simulink model "WallModel"  (R2024a)
settings: Solver=daessc  StartTime=0.0  StopTime=12*3600  FixedStep=3600  MaxStep=3  RelTol=1e-3  AbsTol=1e-3
PreLoadFcn:
  | WallModelParams
values from neighbouring files (symbols this model uses):
  roomHeight = 5    [WallModelParams.m]
undefined symbols (not defined in the file or in its folder): flow, wall, win
libraries: fl_lib x67, nesl_utility x2
CloseFcn:
  | clear flow out roomHeight wall win
settings Model: Creator=vikrants  LastModifiedBy=vikrants
settings SolverCC: AutoScaleAbsTol=off  AlgebraicLoopSolver=TrustRegion  MaxZcPerStep=1
settings DebuggingCC: UnconnectedInputMsg=warning  UnconnectedOutputMsg=warning  UnconnectedLineMsg=warning  SymbolicDimsDataTypeCodeGenerationDiagnostic=none
settings ModelReferenceCC: EnableRefExpFcnMdlSchedulingChecks=on
settings SFSimCC: CustomCodeUndefinedFunction=UseInterfaceOnly
settings RTWCC: GPUComputeCapability=3.5  DLArmComputeVersion=19.05
settings SimscapeCC: SimscapeLogType=all  SimscapeLogSimulationStatistics=on  SimscapeLogDataHistory=10000

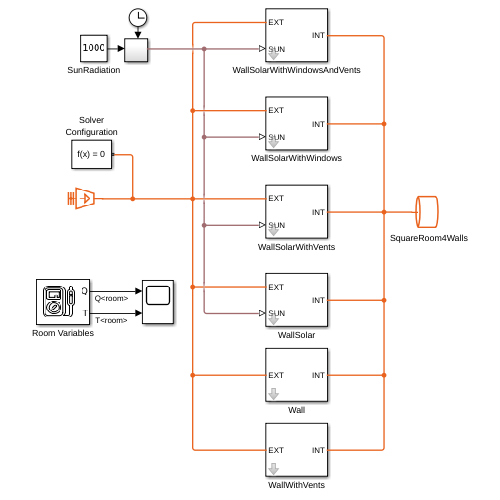
[thumbnail: Simulink's stored preview of the top-level diagram]
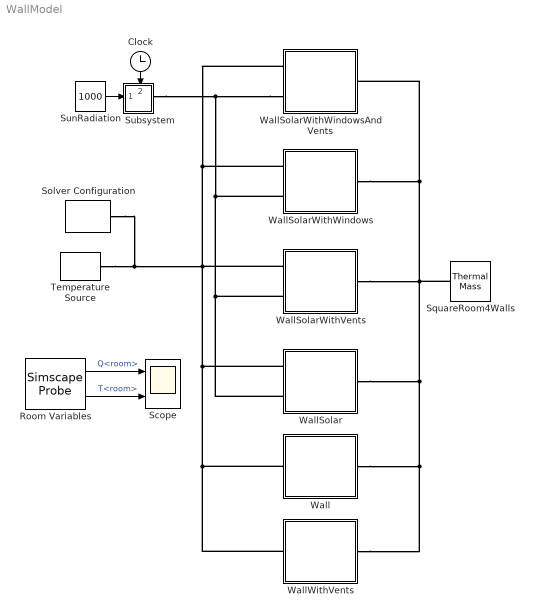
== system WallModel ==
  Clock : Clock
  Room Variables : SimscapeProbe  BoundBlock=26  Variables={Q, T}
  Scope : Scope  NumInputPorts=2
  Solver Configuration : nesl_utility/Solver Configuration  PhysicalDomain=network_engine_domain  SubClassName=solver  LeftPortType=input  RightPortType=generic  Tones=[]  Harmonics=[]  SimulateNoise=off  Profile=off  UseLocalSampling=off  EnableSwitchedLinearOptims=on  FrequencyDomain=off  UseCCode=off  RelTol=0.001  AbsTol=1e-06  MinStep=1e-09  ToWorkspace=off  RevertToSquareIcSolve=off  NumHomotopyIterations=100  PhasorMode=off  PhasorModeNumHarmonics=1  ConsistencySolver=NEWTON_XTOL_AFTER_FTOL  IndexReductionMethod=DerivativeReplacement  DoDC=off  ResidualTolerance=1e-09  ConsistencyTolSource=GLOBAL  ConsistencyAbsTol=0.001  ConsistencyRelTol=0.001  ConsistencyTolFactor=0.001  UseLocalSolver=off  LocalSolverChoice=NE_BACKWARD_EULER_ADVANCER  ResolveIndetEquations=on  FunctionEvalNumThread=1  LocalSolverSampleTime=0.001  DoFixedCost=off  MaxNonlinIter=3  MaxModeIter=2  ComputeImpulses=off  ImpulseIterations=2  LinearAlgebra=auto  LinearAlgebraNumThread=0  EquationFormulation=NE_TIME_EF  DelaysMemoryBudget=1024  AutomaticFiltering=on  FilteringTimeConstant=0.001  PartitionStorageMethod=AS_NEEDED  PartitionMemoryBudget=1024  PartitionMethod=ROBUST  MultibodyUseLocalSolver=off  MultibodyLocalSolverChoice=ODE1  MultibodyLocalSolverSampleTime=0.001
  SquareRoom4Walls : fl_lib/Thermal/Thermal Elements/Thermal Mass  mass_type=foundation.enum.constant_variable.constant  mass=((wall.area+win.area)/roomHeight)^2*flow.airDen kg  sp_heat=flow.airCp J/(K*kg)  mass_min=1e-6 kg  num_ports=foundation.enum.numPorts2.one  m_specify=off  m_priority=High  m=1 kg  m_nominal_specify=off  m_nominal_value=1  m_nominal_unit=kg  T_specify=on  T_priority=High  T=flow.iniT K  T_nominal_specify=off  T_nominal_value=1  T_nominal_unit=K  Q_specify=off  Q_priority=None  Q=0 W  Q_nominal_specify=off  Q_nominal_value=1  Q_nominal_unit=W
  Subsystem : Subsystem
      settings: PortSchema="{\"entries\":[{\"content\":{\"sides\":[{\"content\":{\"connectorIds\":[\"In1\"]},\"type\":\"ConnectorPlacement.EquallySpacedRectSide\",\"uuid\":\"3d46a215-694f-4d20-bc42-8059ad6c23bd\"},{\"content\":{\"connectorIds\":[\"RConn1\"],\"side\":\"RIGHT\"},\"type\":\"ConnectorPlacement.EquallySpacedRectSide\",\"uuid\":\"4734f55e-0044-4fb6-ae62-80969ebadacf\"},{\"content\":{\"connectorIds\":[\"In2\"],\"side\":\"TOP\"},\"type\":\"ConnectorPlacement.EquallySpacedRectSide\",\"uuid\":\"f13755de-7156-4054-ad92-dbe96d889caf\"}]},\"type\":\"ConnectorPlacement.EquallySpacedConnector\",\"uuid\":\"e23b6fdc-de89-4593-96e6-8ffafb2d38ae\"}],\"packageUris\":[\"http://schema.mathworks.com/mf0/Connector/R2020b\"],\"version\":\"1.0\"}"
  SunRadiation : Constant  Value=1000
  Temperature Source : fl_lib/Thermal/Thermal Sources/Temperature Source  temperature=300 K
  Wall : Subsystem  mask{wallArea=wall.area, wallThickness=wall.thickness, wallMaterialMass=wall.mass, wallMaterialCp=wall.Cp, wallThermalK=wall.K, wallAbsorptivity=wall.absorp, extToWallHTC=flow.htc.ext, intToRoomHTC=flow.htc.int, wallTemperature=flow.iniT}
      mask prompts: wallArea "Wall area"; wallThickness "Wall thickness"; wallMaterialMass "Wall material mass"; wallMaterialCp "Wall material heat capacity"; wallThermalK "Wall thermal conductivity"; wallAbsorptivity "Wall absorptivity"; extToWallHTC "Effective heat transfer coefficient from ambient to wall surface"; intToRoomHTC "Effective heat transfer coefficient from internal surface to the room"; wallTemperature "Wall initial temperature"
      mask DialogControl DescTextVar Prompt: Use this custom component to specify the wall heat transfer into a room.
      mask DialogControl Parameters Prompt: Parameters
  WallSolar : Subsystem  mask{wallArea=wall.area, wallThickness=wall.thickness, wallMaterialMass=wall.mass, wallMaterialCp=wall.Cp, wallThermalK=wall.K, wallAbsorptivity=wall.absorp, extToWallHTC=flow.htc.ext, intToRoomHTC=flow.htc.int, wallTemperature=flow.iniT}
      mask prompts: wallArea "Wall area"; wallThickness "Wall thickness"; wallMaterialMass "Wall material mass"; wallMaterialCp "Wall material heat capacity"; wallThermalK "Wall thermal conductivity"; wallAbsorptivity "Wall absorptivity"; extToWallHTC "Effective heat transfer coefficient from ambient to wall surface"; intToRoomHTC "Effective heat transfer coefficient from internal surface to the room"; wallTemperature "Wall initial temperature"
      mask DialogControl DescTextVar Prompt: Use this custom component to specify the wall heat transfer into a room.
      mask DialogControl Parameters Prompt: Parameters
  WallSolarWithVents : Subsystem  mask{wallArea=wall.area, wallThickness=wall.thickness, wallMaterialMass=wall.mass, wallMaterialCp=wall.Cp, wallThermalK=wall.K, wallAbsorptivity=wall.absorp, ventArea=flow.vent.area, extToWallHTC=flow.htc.ext, intToRoomHTC=flow.htc.int, wallTemperature=flow.iniT}
      mask prompts: wallArea "Wall area"; wallThickness "Wall thickness"; wallMaterialMass "Wall material mass"; wallMaterialCp "Wall material heat capacity"; wallThermalK "Wall thermal conductivity"; wallAbsorptivity "Wall absorptivity"; ventArea "Vent area"; extToWallHTC "Effective heat transfer coefficient from ambient to wall surface"; intToRoomHTC "Effective heat transfer coefficient from internal surface to the room"; wallTemperature "Wall initial temperature"
      mask DialogControl DescTextVar Prompt: Use this custom component to specify the wall and assicated heat transfer into a room. You must specify the wall and window material properties along with the vent size.
      mask DialogControl Parameters Prompt: Parameters
  WallSolarWithWindows : Subsystem  mask{winArea=win.area, winThickness=win.thickness, winMaterialMass=win.mass, winMaterialCp=win.Cp, winThermalK=win.K, winAbsorptivity=win.absorp, winTransmissivity=win.trans, wallArea=wall.area, wallThickness=wall.thickness, wallMaterialMass=wall.mass, wallMaterialCp=wall.Cp, wallThermalK=wall.K, wallAbsorptivity=wall.absorp, extToWallHTC=flow.htc.ext, intToRoomHTC=flow.htc.int, wallTemperature=flow.iniT, winTemperature=flow.iniT}
      mask prompts: winArea "Window area"; winThickness "Window thickness"; winMaterialMass "Window material mass"; winMaterialCp "Window material heat capacity"; winThermalK "Window thermal conductivity"; winAbsorptivity "Window Absorptivity"; winTransmissivity "Window transmissivity"; wallArea "Wall area"; wallThickness "Wall thickness"; wallMaterialMass "Wall material mass"; wallMaterialCp "Wall material heat capacity"; wallThermalK "Wall thermal conductivity"; wallAbsorptivity "Wall absorptivity"; extToWallHTC "Effective heat transfer coefficient from ambient to wall surface"; intToRoomHTC "Effective heat transfer coefficient from internal surface to the room"; wallTemperature "Wall initial temperature"; winTemperature "Window initial temperature"
      mask DialogControl DescTextVar Prompt: Use this custom component to specify the wall and assicated heat transfer into a room. You must specify the wall and window material properties.
      mask DialogControl Parameters Prompt: Parameters
  WallSolarWithWindowsAndVents : Subsystem  mask{winArea=win.area, winThickness=win.thickness, winMaterialMass=win.mass, winMaterialCp=win.Cp, winThermalK=win.K, winAbsorptivity=win.absorp, winTransmissivity=win.trans, wallArea=wall.area, wallThickness=wall.thickness, wallMaterialMass=wall.mass, wallMaterialCp=wall.Cp, wallThermalK=wall.K, wallAbsorptivity=wall.absorp, ventArea=flow.vent.area, extToWallHTC=flow.htc.ext, intToRoomHTC=flow.htc.int, wallTemperature=flow.iniT, winTemperature=flow.iniT}
      mask prompts: winArea "Window area"; winThickness "Window thickness"; winMaterialMass "Window material mass"; winMaterialCp "Window material heat capacity"; winThermalK "Window thermal conductivity"; winAbsorptivity "Window Absorptivity"; winTransmissivity "Window transmissivity"; wallArea "Wall area"; wallThickness "Wall thickness"; wallMaterialMass "Wall material mass"; wallMaterialCp "Wall material heat capacity"; wallThermalK "Wall thermal conductivity"; wallAbsorptivity "Wall absorptivity"; ventArea "Vent area"; extToWallHTC "Effective heat transfer coefficient from ambient to wall surface"; intToRoomHTC "Effective heat transfer coefficient from internal surface to the room"; wallTemperature "Wall initial temperature"; winTemperature "Window initial temperature"
      mask DialogControl DescTextVar Prompt: Use this custom component to specify the wall and assicated heat transfer into a room. You must specify the wall and window material properties along with the vent size.
      mask DialogControl Parameters Prompt: Parameters
  WallWithVents : Subsystem  mask{wallArea=wall.area, wallThickness=wall.thickness, wallMaterialMass=wall.mass, wallMaterialCp=wall.Cp, wallThermalK=wall.K, ventArea=flow.vent.area, extToWallHTC=flow.htc.ext, intToRoomHTC=flow.htc.int, wallTemperature=flow.iniT}
      mask prompts: wallArea "Wall area"; wallThickness "Wall thickness"; wallMaterialMass "Wall material mass"; wallMaterialCp "Wall material heat capacity"; wallThermalK "Wall thermal conductivity"; ventArea "Vent area"; extToWallHTC "Effective heat transfer coefficient from ambient to wall surface"; intToRoomHTC "Effective heat transfer coefficient from internal surface to the room"; wallTemperature "Wall initial temperature"
      mask DialogControl DescTextVar Prompt: Use this custom component to specify the wall and assicated heat transfer into a room. You must specify the wall and window material properties along with the vent size.
      mask DialogControl Parameters Prompt: Parameters
  wires:
  Room Variables/2 -> Scope/2  "T<room>"
  Room Variables/1 -> Scope/1  "Q<room>"
  Clock/1 -> Subsystem/2(" ")
  SunRadiation/1 -> Subsystem/1("  ")
  connections:
  SquareRoom4Walls/LConn1 -- WallSolarWithWindowsAndVents/RConn1 -- WallSolarWithWindows/RConn1 -- WallWithVents/RConn1 -- Wall/RConn1 -- WallSolar/RConn1 -- WallSolarWithVents/RConn1
  WallSolarWithWindowsAndVents/LConn2 -- WallSolar/LConn2 -- WallSolarWithVents/LConn2 -- WallSolarWithWindows/LConn2 -- Subsystem/RConn1
  Temperature Source/LConn1 -- Solver Configuration/RConn1 -- WallSolarWithWindowsAndVents/LConn1 -- WallSolarWithWindows/LConn1 -- WallWithVents/LConn1 -- Wall/LConn1 -- WallSolar/LConn1 -- WallSolarWithVents/LConn1

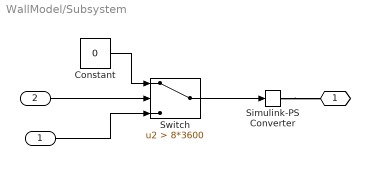
== system WallModel/Subsystem ==
  "  " : Inport
  " " : Inport  Port=2
  Constant : Constant  Value=0
  Simulink-PS Converter : nesl_utility/Simulink-PS Converter  PhysicalDomain=network_engine_domain  SubClassName=ps_input  LeftPortType=input  RightPortType=output  PseudoPeriodic=off  Frequencies=[]  NoiseDistribution=none  NoiseParameters=[]  Unit=W/m^2  AffineConversion=off  FilteringAndDerivatives=filter  SimscapeFilterOrder=1  InputFilterTimeConstant=0.001  UdotUserProvided=0
  Switch : Switch  Criteria=u2 > Threshold  Threshold=8*3600  SaturateOnIntegerOverflow=off  InputSameDT=off
  "   " : PMIOPort  Side=Right
  wires:
  Switch/1 -> Simulink-PS Converter/1
  Constant/1 -> Switch/1
  " "/1 -> Switch/2
  "  "/1 -> Switch/3
  connections:
  Simulink-PS Converter/RConn1 -- "   "/RConn1

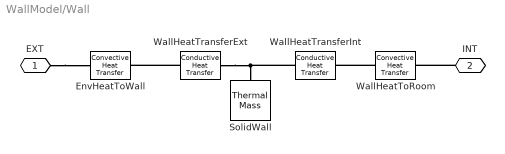
== system WallModel/Wall ==
  EnvHeatToWall : fl_lib/Thermal/Thermal Elements/Convective Heat Transfer  thermal_type=foundation.enum.constant_variable.constant  area=wallArea m^2  heat_tr_coeff=extToWallHTC W/(K*m^2)  min_heat_tr_coeff=1e-3 W/(K*m^2)  T_specify=off  T_priority=None  T=0 K  T_nominal_specify=off  T_nominal_value=1  T_nominal_unit=K  Q_specify=off  Q_priority=None  Q=0 W  Q_nominal_specify=off  Q_nominal_value=1  Q_nominal_unit=W
  SolidWall : fl_lib/Thermal/Thermal Elements/Thermal Mass  mass_type=foundation.enum.constant_variable.constant  mass=wallMaterialMass kg  sp_heat=wallMaterialCp J/(K*kg)  mass_min=1e-6 kg  num_ports=foundation.enum.numPorts2.one  m_specify=off  m_priority=High  m=1 kg  m_nominal_specify=off  m_nominal_value=1  m_nominal_unit=kg  T_specify=on  T_priority=High  T=wallTemperature K  T_nominal_specify=off  T_nominal_value=1  T_nominal_unit=K  Q_specify=off  Q_priority=None  Q=0 W  Q_nominal_specify=off  Q_nominal_value=1  Q_nominal_unit=W
  WallHeatToRoom : fl_lib/Thermal/Thermal Elements/Convective Heat Transfer  thermal_type=foundation.enum.constant_variable.constant  area=wallArea m^2  heat_tr_coeff=intToRoomHTC W/(K*m^2)  min_heat_tr_coeff=1e-3 W/(K*m^2)  T_specify=off  T_priority=None  T=0 K  T_nominal_specify=off  T_nominal_value=1  T_nominal_unit=K  Q_specify=off  Q_priority=None  Q=0 W  Q_nominal_specify=off  Q_nominal_value=1  Q_nominal_unit=W
  WallHeatTransferExt : fl_lib/Thermal/Thermal Elements/Conductive Heat Transfer  thermal_type=foundation.enum.ConstantVariableTabulated.Constant  wall_geometry=foundation.enum.ConductionWallGeometry.Planar  area=wallArea m^2  thickness=wallThickness m  d_in=0.05 m  d_out=0.1 m  L=1 m  th_cond_min=10 W/(K*m)  th_cond=wallThermalK W/(K*m)  th_cond_TLU=[413, 401, 392, 383, 371, 357, 342] W/(K*m)  temp_TLU=[200, 273, 400, 600, 800, 1000, 1200] K  T_specify=off  T_priority=None  T=0 K  T_nominal_specify=off  T_nominal_value=1  T_nominal_unit=K  Q_specify=off  Q_priority=None  Q=0 W  Q_nominal_specify=off  Q_nominal_value=1  Q_nominal_unit=W
  WallHeatTransferInt : fl_lib/Thermal/Thermal Elements/Conductive Heat Transfer  thermal_type=foundation.enum.ConstantVariableTabulated.Constant  wall_geometry=foundation.enum.ConductionWallGeometry.Planar  area=wallArea m^2  thickness=wallThickness m  d_in=0.05 m  d_out=0.1 m  L=1 m  th_cond_min=10 W/(K*m)  th_cond=wallThermalK W/(K*m)  th_cond_TLU=[413, 401, 392, 383, 371, 357, 342] W/(K*m)  temp_TLU=[200, 273, 400, 600, 800, 1000, 1200] K  T_specify=off  T_priority=None  T=0 K  T_nominal_specify=off  T_nominal_value=1  T_nominal_unit=K  Q_specify=off  Q_priority=None  Q=0 W  Q_nominal_specify=off  Q_nominal_value=1  Q_nominal_unit=W
  EXT : PMIOPort  Side=Left
  INT : PMIOPort  Port=2  Side=Right
  connections:
  WallHeatToRoom/LConn1 -- WallHeatTransferInt/RConn1
  INT/RConn1 -- WallHeatToRoom/RConn1
  EXT/RConn1 -- EnvHeatToWall/LConn1
  WallHeatTransferExt/LConn1 -- EnvHeatToWall/RConn1
  WallHeatTransferExt/RConn1 -- WallHeatTransferInt/LConn1 -- SolidWall/LConn1

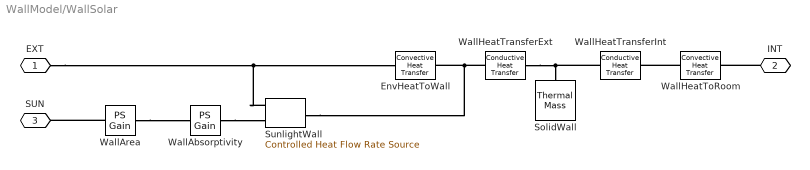
== system WallModel/WallSolar ==
  EnvHeatToWall : fl_lib/Thermal/Thermal Elements/Convective Heat Transfer  thermal_type=foundation.enum.constant_variable.constant  area=wallArea m^2  heat_tr_coeff=extToWallHTC W/(K*m^2)  min_heat_tr_coeff=1e-3 W/(K*m^2)  T_specify=off  T_priority=None  T=0 K  T_nominal_specify=off  T_nominal_value=1  T_nominal_unit=K  Q_specify=off  Q_priority=None  Q=0 W  Q_nominal_specify=off  Q_nominal_value=1  Q_nominal_unit=W
  SolidWall : fl_lib/Thermal/Thermal Elements/Thermal Mass  mass_type=foundation.enum.constant_variable.constant  mass=wallMaterialMass kg  sp_heat=wallMaterialCp J/(K*kg)  mass_min=1e-6 kg  num_ports=foundation.enum.numPorts2.one  m_specify=off  m_priority=High  m=1 kg  m_nominal_specify=off  m_nominal_value=1  m_nominal_unit=kg  T_specify=on  T_priority=High  T=wallTemperature K  T_nominal_specify=off  T_nominal_value=1  T_nominal_unit=K  Q_specify=off  Q_priority=None  Q=0 W  Q_nominal_specify=off  Q_nominal_value=1  Q_nominal_unit=W
  SunlightWall : fl_lib/Thermal/Thermal Sources/Controlled Heat Flow Rate Source
  WallAbsorptivity : fl_lib/Physical Signals/Functions/PS Gain  gain=wallAbsorptivity
  WallArea : fl_lib/Physical Signals/Functions/PS Gain  gain=wallArea m^2
  WallHeatToRoom : fl_lib/Thermal/Thermal Elements/Convective Heat Transfer  thermal_type=foundation.enum.constant_variable.constant  area=wallArea m^2  heat_tr_coeff=intToRoomHTC W/(K*m^2)  min_heat_tr_coeff=1e-3 W/(K*m^2)  T_specify=off  T_priority=None  T=0 K  T_nominal_specify=off  T_nominal_value=1  T_nominal_unit=K  Q_specify=off  Q_priority=None  Q=0 W  Q_nominal_specify=off  Q_nominal_value=1  Q_nominal_unit=W
  WallHeatTransferExt : fl_lib/Thermal/Thermal Elements/Conductive Heat Transfer  thermal_type=foundation.enum.ConstantVariableTabulated.Constant  wall_geometry=foundation.enum.ConductionWallGeometry.Planar  area=wallArea m^2  thickness=wallThickness m  d_in=0.05 m  d_out=0.1 m  L=1 m  th_cond_min=10 W/(K*m)  th_cond=wallThermalK W/(K*m)  th_cond_TLU=[413, 401, 392, 383, 371, 357, 342] W/(K*m)  temp_TLU=[200, 273, 400, 600, 800, 1000, 1200] K  T_specify=off  T_priority=None  T=0 K  T_nominal_specify=off  T_nominal_value=1  T_nominal_unit=K  Q_specify=off  Q_priority=None  Q=0 W  Q_nominal_specify=off  Q_nominal_value=1  Q_nominal_unit=W
  WallHeatTransferInt : fl_lib/Thermal/Thermal Elements/Conductive Heat Transfer  thermal_type=foundation.enum.ConstantVariableTabulated.Constant  wall_geometry=foundation.enum.ConductionWallGeometry.Planar  area=wallArea m^2  thickness=wallThickness m  d_in=0.05 m  d_out=0.1 m  L=1 m  th_cond_min=10 W/(K*m)  th_cond=wallThermalK W/(K*m)  th_cond_TLU=[413, 401, 392, 383, 371, 357, 342] W/(K*m)  temp_TLU=[200, 273, 400, 600, 800, 1000, 1200] K  T_specify=off  T_priority=None  T=0 K  T_nominal_specify=off  T_nominal_value=1  T_nominal_unit=K  Q_specify=off  Q_priority=None  Q=0 W  Q_nominal_specify=off  Q_nominal_value=1  Q_nominal_unit=W
  EXT : PMIOPort  Side=Left
  INT : PMIOPort  Port=2  Side=Right
  SUN : PMIOPort  Port=3  Side=Left
  connections:
  WallHeatToRoom/LConn1 -- WallHeatTransferInt/RConn1
  INT/RConn1 -- WallHeatToRoom/RConn1
  SunlightWall/RConn2 -- EXT/RConn1 -- EnvHeatToWall/LConn1
  WallHeatTransferExt/LConn1 -- SunlightWall/LConn1 -- EnvHeatToWall/RConn1
  WallHeatTransferExt/RConn1 -- WallHeatTransferInt/LConn1 -- SolidWall/LConn1
  WallAbsorptivity/RConn1 -- SunlightWall/RConn1
  WallArea/LConn1 -- SUN/RConn1
  WallArea/RConn1 -- WallAbsorptivity/LConn1

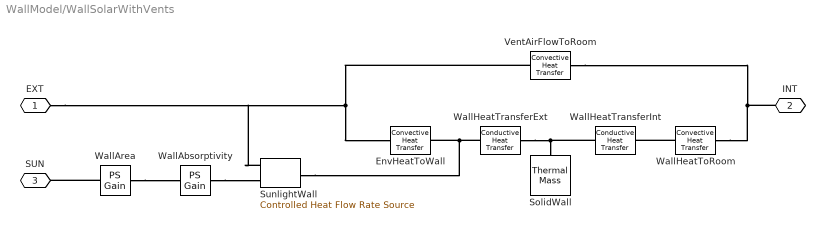
== system WallModel/WallSolarWithVents ==
  EnvHeatToWall : fl_lib/Thermal/Thermal Elements/Convective Heat Transfer  thermal_type=foundation.enum.constant_variable.constant  area=wallArea m^2  heat_tr_coeff=extToWallHTC W/(K*m^2)  min_heat_tr_coeff=1e-3 W/(K*m^2)  T_specify=off  T_priority=None  T=0 K  T_nominal_specify=off  T_nominal_value=1  T_nominal_unit=K  Q_specify=off  Q_priority=None  Q=0 W  Q_nominal_specify=off  Q_nominal_value=1  Q_nominal_unit=W
  SolidWall : fl_lib/Thermal/Thermal Elements/Thermal Mass  mass_type=foundation.enum.constant_variable.constant  mass=wallMaterialMass kg  sp_heat=wallMaterialCp J/(K*kg)  mass_min=1e-6 kg  num_ports=foundation.enum.numPorts2.one  m_specify=off  m_priority=High  m=1 kg  m_nominal_specify=off  m_nominal_value=1  m_nominal_unit=kg  T_specify=on  T_priority=High  T=wallTemperature K  T_nominal_specify=off  T_nominal_value=1  T_nominal_unit=K  Q_specify=off  Q_priority=None  Q=0 W  Q_nominal_specify=off  Q_nominal_value=1  Q_nominal_unit=W
  SunlightWall : fl_lib/Thermal/Thermal Sources/Controlled Heat Flow Rate Source
  VentAirFlowToRoom : fl_lib/Thermal/Thermal Elements/Convective Heat Transfer  thermal_type=foundation.enum.constant_variable.constant  area=ventArea m^2  heat_tr_coeff=extToWallHTC W/(K*m^2)  min_heat_tr_coeff=1e-3 W/(K*m^2)  T_specify=off  T_priority=None  T=0 K  T_nominal_specify=off  T_nominal_value=1  T_nominal_unit=K  Q_specify=off  Q_priority=None  Q=0 W  Q_nominal_specify=off  Q_nominal_value=1  Q_nominal_unit=W
  WallAbsorptivity : fl_lib/Physical Signals/Functions/PS Gain  gain=wallAbsorptivity
  WallArea : fl_lib/Physical Signals/Functions/PS Gain  gain=wallArea m^2
  WallHeatToRoom : fl_lib/Thermal/Thermal Elements/Convective Heat Transfer  thermal_type=foundation.enum.constant_variable.constant  area=wallArea m^2  heat_tr_coeff=intToRoomHTC W/(K*m^2)  min_heat_tr_coeff=1e-3 W/(K*m^2)  T_specify=off  T_priority=None  T=0 K  T_nominal_specify=off  T_nominal_value=1  T_nominal_unit=K  Q_specify=off  Q_priority=None  Q=0 W  Q_nominal_specify=off  Q_nominal_value=1  Q_nominal_unit=W
  WallHeatTransferExt : fl_lib/Thermal/Thermal Elements/Conductive Heat Transfer  thermal_type=foundation.enum.ConstantVariableTabulated.Constant  wall_geometry=foundation.enum.ConductionWallGeometry.Planar  area=wallArea m^2  thickness=wallThickness m  d_in=0.05 m  d_out=0.1 m  L=1 m  th_cond_min=10 W/(K*m)  th_cond=wallThermalK W/(K*m)  th_cond_TLU=[413, 401, 392, 383, 371, 357, 342] W/(K*m)  temp_TLU=[200, 273, 400, 600, 800, 1000, 1200] K  T_specify=off  T_priority=None  T=0 K  T_nominal_specify=off  T_nominal_value=1  T_nominal_unit=K  Q_specify=off  Q_priority=None  Q=0 W  Q_nominal_specify=off  Q_nominal_value=1  Q_nominal_unit=W
  WallHeatTransferInt : fl_lib/Thermal/Thermal Elements/Conductive Heat Transfer  thermal_type=foundation.enum.ConstantVariableTabulated.Constant  wall_geometry=foundation.enum.ConductionWallGeometry.Planar  area=wallArea m^2  thickness=wallThickness m  d_in=0.05 m  d_out=0.1 m  L=1 m  th_cond_min=10 W/(K*m)  th_cond=wallThermalK W/(K*m)  th_cond_TLU=[413, 401, 392, 383, 371, 357, 342] W/(K*m)  temp_TLU=[200, 273, 400, 600, 800, 1000, 1200] K  T_specify=off  T_priority=None  T=0 K  T_nominal_specify=off  T_nominal_value=1  T_nominal_unit=K  Q_specify=off  Q_priority=None  Q=0 W  Q_nominal_specify=off  Q_nominal_value=1  Q_nominal_unit=W
  EXT : PMIOPort  Side=Left
  INT : PMIOPort  Port=2  Side=Right
  SUN : PMIOPort  Port=3  Side=Left
  connections:
  WallHeatToRoom/LConn1 -- WallHeatTransferInt/RConn1
  VentAirFlowToRoom/RConn1 -- WallHeatToRoom/RConn1 -- INT/RConn1
  VentAirFlowToRoom/LConn1 -- EXT/RConn1 -- SunlightWall/RConn2 -- EnvHeatToWall/LConn1
  WallHeatTransferExt/LConn1 -- SunlightWall/LConn1 -- EnvHeatToWall/RConn1
  WallHeatTransferExt/RConn1 -- WallHeatTransferInt/LConn1 -- SolidWall/LConn1
  WallAbsorptivity/RConn1 -- SunlightWall/RConn1
  WallArea/LConn1 -- SUN/RConn1
  WallArea/RConn1 -- WallAbsorptivity/LConn1

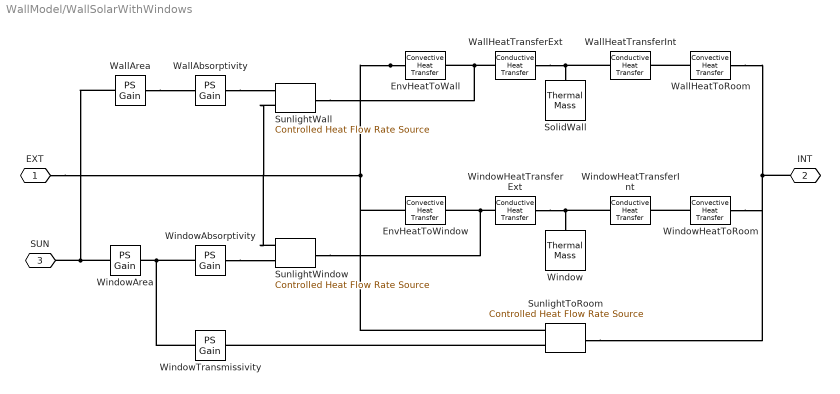
== system WallModel/WallSolarWithWindows ==
  EnvHeatToWall : fl_lib/Thermal/Thermal Elements/Convective Heat Transfer  thermal_type=foundation.enum.constant_variable.constant  area=wallArea m^2  heat_tr_coeff=extToWallHTC W/(K*m^2)  min_heat_tr_coeff=1e-3 W/(K*m^2)  T_specify=off  T_priority=None  T=0 K  T_nominal_specify=off  T_nominal_value=1  T_nominal_unit=K  Q_specify=off  Q_priority=None  Q=0 W  Q_nominal_specify=off  Q_nominal_value=1  Q_nominal_unit=W
  EnvHeatToWindow : fl_lib/Thermal/Thermal Elements/Convective Heat Transfer  thermal_type=foundation.enum.constant_variable.constant  area=winArea m^2  heat_tr_coeff=extToWallHTC W/(K*m^2)  min_heat_tr_coeff=1e-3 W/(K*m^2)  T_specify=off  T_priority=None  T=0 K  T_nominal_specify=off  T_nominal_value=1  T_nominal_unit=K  Q_specify=off  Q_priority=None  Q=0 W  Q_nominal_specify=off  Q_nominal_value=1  Q_nominal_unit=W
  SolidWall : fl_lib/Thermal/Thermal Elements/Thermal Mass  mass_type=foundation.enum.constant_variable.constant  mass=wallMaterialMass kg  sp_heat=wallMaterialCp J/(K*kg)  mass_min=1e-6 kg  num_ports=foundation.enum.numPorts2.one  m_specify=off  m_priority=High  m=1 kg  m_nominal_specify=off  m_nominal_value=1  m_nominal_unit=kg  T_specify=on  T_priority=High  T=wallTemperature K  T_nominal_specify=off  T_nominal_value=1  T_nominal_unit=K  Q_specify=off  Q_priority=None  Q=0 W  Q_nominal_specify=off  Q_nominal_value=1  Q_nominal_unit=W
  SunlightToRoom : fl_lib/Thermal/Thermal Sources/Controlled Heat Flow Rate Source
  SunlightWall : fl_lib/Thermal/Thermal Sources/Controlled Heat Flow Rate Source
  SunlightWindow : fl_lib/Thermal/Thermal Sources/Controlled Heat Flow Rate Source
  WallAbsorptivity : fl_lib/Physical Signals/Functions/PS Gain  gain=wallAbsorptivity
  WallArea : fl_lib/Physical Signals/Functions/PS Gain  gain=wallArea m^2
  WallHeatToRoom : fl_lib/Thermal/Thermal Elements/Convective Heat Transfer  thermal_type=foundation.enum.constant_variable.constant  area=wallArea m^2  heat_tr_coeff=intToRoomHTC W/(K*m^2)  min_heat_tr_coeff=1e-3 W/(K*m^2)  T_specify=off  T_priority=None  T=0 K  T_nominal_specify=off  T_nominal_value=1  T_nominal_unit=K  Q_specify=off  Q_priority=None  Q=0 W  Q_nominal_specify=off  Q_nominal_value=1  Q_nominal_unit=W
  WallHeatTransferExt : fl_lib/Thermal/Thermal Elements/Conductive Heat Transfer  thermal_type=foundation.enum.ConstantVariableTabulated.Constant  wall_geometry=foundation.enum.ConductionWallGeometry.Planar  area=wallArea m^2  thickness=wallThickness m  d_in=0.05 m  d_out=0.1 m  L=1 m  th_cond_min=10 W/(K*m)  th_cond=wallThermalK W/(K*m)  th_cond_TLU=[413, 401, 392, 383, 371, 357, 342] W/(K*m)  temp_TLU=[200, 273, 400, 600, 800, 1000, 1200] K  T_specify=off  T_priority=None  T=0 K  T_nominal_specify=off  T_nominal_value=1  T_nominal_unit=K  Q_specify=off  Q_priority=None  Q=0 W  Q_nominal_specify=off  Q_nominal_value=1  Q_nominal_unit=W
  WallHeatTransferInt : fl_lib/Thermal/Thermal Elements/Conductive Heat Transfer  thermal_type=foundation.enum.ConstantVariableTabulated.Constant  wall_geometry=foundation.enum.ConductionWallGeometry.Planar  area=wallArea m^2  thickness=wallThickness m  d_in=0.05 m  d_out=0.1 m  L=1 m  th_cond_min=10 W/(K*m)  th_cond=wallThermalK W/(K*m)  th_cond_TLU=[413, 401, 392, 383, 371, 357, 342] W/(K*m)  temp_TLU=[200, 273, 400, 600, 800, 1000, 1200] K  T_specify=off  T_priority=None  T=0 K  T_nominal_specify=off  T_nominal_value=1  T_nominal_unit=K  Q_specify=off  Q_priority=None  Q=0 W  Q_nominal_specify=off  Q_nominal_value=1  Q_nominal_unit=W
  Window : fl_lib/Thermal/Thermal Elements/Thermal Mass  mass_type=foundation.enum.constant_variable.constant  mass=winMaterialMass kg  sp_heat=winMaterialCp J/(K*kg)  mass_min=1e-6 kg  num_ports=foundation.enum.numPorts2.one  m_specify=off  m_priority=High  m=1 kg  m_nominal_specify=off  m_nominal_value=1  m_nominal_unit=kg  T_specify=on  T_priority=High  T=winTemperature K  T_nominal_specify=off  T_nominal_value=1  T_nominal_unit=K  Q_specify=off  Q_priority=None  Q=0 W  Q_nominal_specify=off  Q_nominal_value=1  Q_nominal_unit=W
  WindowAbsorptivity : fl_lib/Physical Signals/Functions/PS Gain  gain=winAbsorptivity
  WindowArea : fl_lib/Physical Signals/Functions/PS Gain  gain=winArea m^2
  WindowHeatToRoom : fl_lib/Thermal/Thermal Elements/Convective Heat Transfer  thermal_type=foundation.enum.constant_variable.constant  area=winArea m^2  heat_tr_coeff=intToRoomHTC W/(K*m^2)  min_heat_tr_coeff=1e-3 W/(K*m^2)  T_specify=off  T_priority=None  T=0 K  T_nominal_specify=off  T_nominal_value=1  T_nominal_unit=K  Q_specify=off  Q_priority=None  Q=0 W  Q_nominal_specify=off  Q_nominal_value=1  Q_nominal_unit=W
  WindowHeatTransferExt : fl_lib/Thermal/Thermal Elements/Conductive Heat Transfer  thermal_type=foundation.enum.ConstantVariableTabulated.Constant  wall_geometry=foundation.enum.ConductionWallGeometry.Planar  area=winArea m^2  thickness=winThickness m  d_in=0.05 m  d_out=0.1 m  L=1 m  th_cond_min=10 W/(K*m)  th_cond=winThermalK W/(K*m)  th_cond_TLU=[413, 401, 392, 383, 371, 357, 342] W/(K*m)  temp_TLU=[200, 273, 400, 600, 800, 1000, 1200] K  T_specify=off  T_priority=None  T=0 K  T_nominal_specify=off  T_nominal_value=1  T_nominal_unit=K  Q_specify=off  Q_priority=None  Q=0 W  Q_nominal_specify=off  Q_nominal_value=1  Q_nominal_unit=W
  WindowHeatTransferInt : fl_lib/Thermal/Thermal Elements/Conductive Heat Transfer  thermal_type=foundation.enum.ConstantVariableTabulated.Constant  wall_geometry=foundation.enum.ConductionWallGeometry.Planar  area=winArea m^2  thickness=winThickness m  d_in=0.05 m  d_out=0.1 m  L=1 m  th_cond_min=10 W/(K*m)  th_cond=winThermalK W/(K*m)  th_cond_TLU=[413, 401, 392, 383, 371, 357, 342] W/(K*m)  temp_TLU=[200, 273, 400, 600, 800, 1000, 1200] K  T_specify=off  T_priority=None  T=0 K  T_nominal_specify=off  T_nominal_value=1  T_nominal_unit=K  Q_specify=off  Q_priority=None  Q=0 W  Q_nominal_specify=off  Q_nominal_value=1  Q_nominal_unit=W
  WindowTransmissivity : fl_lib/Physical Signals/Functions/PS Gain  gain=winTransmissivity
  EXT : PMIOPort  Side=Left
  INT : PMIOPort  Port=2  Side=Right
  SUN : PMIOPort  Port=3  Side=Left
  connections:
  WallHeatToRoom/LConn1 -- WallHeatTransferInt/RConn1
  WindowHeatToRoom/LConn1 -- WindowHeatTransferInt/RConn1
  WindowHeatTransferInt/LConn1 -- WindowHeatTransferExt/RConn1 -- Window/LConn1
  INT/RConn1 -- WallHeatToRoom/RConn1 -- SunlightToRoom/LConn1 -- WindowHeatToRoom/RConn1
  EnvHeatToWall/LConn1 -- SunlightWall/RConn2 -- EXT/RConn1 -- SunlightWindow/RConn2 -- EnvHeatToWindow/LConn1 -- SunlightToRoom/RConn2
  WallHeatTransferExt/LConn1 -- SunlightWall/LConn1 -- EnvHeatToWall/RConn1
  WindowHeatTransferExt/LConn1 -- SunlightWindow/LConn1 -- EnvHeatToWindow/RConn1
  WallHeatTransferExt/RConn1 -- WallHeatTransferInt/LConn1 -- SolidWall/LConn1
  WindowAbsorptivity/LConn1 -- WindowTransmissivity/LConn1 -- WindowArea/RConn1
  SunlightToRoom/RConn1 -- WindowTransmissivity/RConn1
  WallAbsorptivity/RConn1 -- SunlightWall/RConn1
  WindowAbsorptivity/RConn1 -- SunlightWindow/RConn1
  WindowArea/LConn1 -- WallArea/LConn1 -- SUN/RConn1
  WallArea/RConn1 -- WallAbsorptivity/LConn1

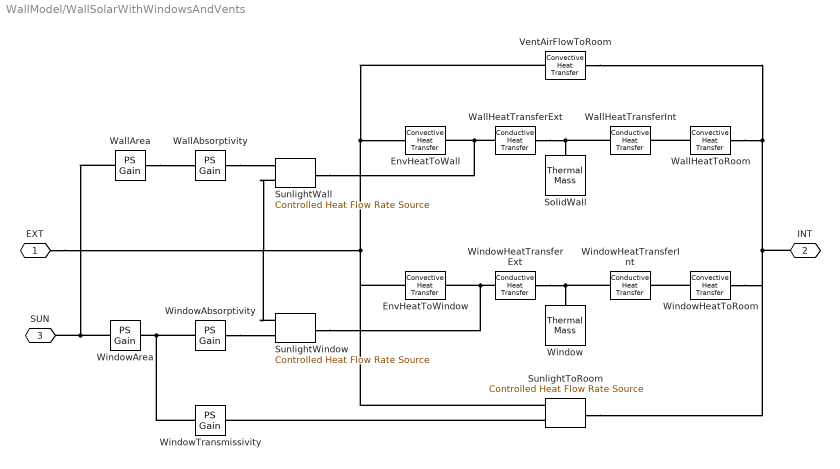
== system WallModel/WallSolarWithWindowsAndVents ==
  EnvHeatToWall : fl_lib/Thermal/Thermal Elements/Convective Heat Transfer  thermal_type=foundation.enum.constant_variable.constant  area=wallArea m^2  heat_tr_coeff=extToWallHTC W/(K*m^2)  min_heat_tr_coeff=1e-3 W/(K*m^2)  T_specify=off  T_priority=None  T=0 K  T_nominal_specify=off  T_nominal_value=1  T_nominal_unit=K  Q_specify=off  Q_priority=None  Q=0 W  Q_nominal_specify=off  Q_nominal_value=1  Q_nominal_unit=W
  EnvHeatToWindow : fl_lib/Thermal/Thermal Elements/Convective Heat Transfer  thermal_type=foundation.enum.constant_variable.constant  area=winArea m^2  heat_tr_coeff=extToWallHTC W/(K*m^2)  min_heat_tr_coeff=1e-3 W/(K*m^2)  T_specify=off  T_priority=None  T=0 K  T_nominal_specify=off  T_nominal_value=1  T_nominal_unit=K  Q_specify=off  Q_priority=None  Q=0 W  Q_nominal_specify=off  Q_nominal_value=1  Q_nominal_unit=W
  SolidWall : fl_lib/Thermal/Thermal Elements/Thermal Mass  mass_type=foundation.enum.constant_variable.constant  mass=wallMaterialMass kg  sp_heat=wallMaterialCp J/(K*kg)  mass_min=1e-6 kg  num_ports=foundation.enum.numPorts2.one  m_specify=off  m_priority=High  m=1 kg  m_nominal_specify=off  m_nominal_value=1  m_nominal_unit=kg  T_specify=on  T_priority=High  T=wallTemperature K  T_nominal_specify=off  T_nominal_value=1  T_nominal_unit=K  Q_specify=off  Q_priority=None  Q=0 W  Q_nominal_specify=off  Q_nominal_value=1  Q_nominal_unit=W
  SunlightToRoom : fl_lib/Thermal/Thermal Sources/Controlled Heat Flow Rate Source
  SunlightWall : fl_lib/Thermal/Thermal Sources/Controlled Heat Flow Rate Source
  SunlightWindow : fl_lib/Thermal/Thermal Sources/Controlled Heat Flow Rate Source
  VentAirFlowToRoom : fl_lib/Thermal/Thermal Elements/Convective Heat Transfer  thermal_type=foundation.enum.constant_variable.constant  area=ventArea m^2  heat_tr_coeff=extToWallHTC W/(K*m^2)  min_heat_tr_coeff=1e-3 W/(K*m^2)  T_specify=off  T_priority=None  T=0 K  T_nominal_specify=off  T_nominal_value=1  T_nominal_unit=K  Q_specify=off  Q_priority=None  Q=0 W  Q_nominal_specify=off  Q_nominal_value=1  Q_nominal_unit=W
  WallAbsorptivity : fl_lib/Physical Signals/Functions/PS Gain  gain=wallAbsorptivity
  WallArea : fl_lib/Physical Signals/Functions/PS Gain  gain=wallArea m^2
  WallHeatToRoom : fl_lib/Thermal/Thermal Elements/Convective Heat Transfer  thermal_type=foundation.enum.constant_variable.constant  area=wallArea m^2  heat_tr_coeff=intToRoomHTC W/(K*m^2)  min_heat_tr_coeff=1e-3 W/(K*m^2)  T_specify=off  T_priority=None  T=0 K  T_nominal_specify=off  T_nominal_value=1  T_nominal_unit=K  Q_specify=off  Q_priority=None  Q=0 W  Q_nominal_specify=off  Q_nominal_value=1  Q_nominal_unit=W
  WallHeatTransferExt : fl_lib/Thermal/Thermal Elements/Conductive Heat Transfer  thermal_type=foundation.enum.ConstantVariableTabulated.Constant  wall_geometry=foundation.enum.ConductionWallGeometry.Planar  area=wallArea m^2  thickness=wallThickness m  d_in=0.05 m  d_out=0.1 m  L=1 m  th_cond_min=10 W/(K*m)  th_cond=wallThermalK W/(K*m)  th_cond_TLU=[413, 401, 392, 383, 371, 357, 342] W/(K*m)  temp_TLU=[200, 273, 400, 600, 800, 1000, 1200] K  T_specify=off  T_priority=None  T=0 K  T_nominal_specify=off  T_nominal_value=1  T_nominal_unit=K  Q_specify=off  Q_priority=None  Q=0 W  Q_nominal_specify=off  Q_nominal_value=1  Q_nominal_unit=W
  WallHeatTransferInt : fl_lib/Thermal/Thermal Elements/Conductive Heat Transfer  thermal_type=foundation.enum.ConstantVariableTabulated.Constant  wall_geometry=foundation.enum.ConductionWallGeometry.Planar  area=wallArea m^2  thickness=wallThickness m  d_in=0.05 m  d_out=0.1 m  L=1 m  th_cond_min=10 W/(K*m)  th_cond=wallThermalK W/(K*m)  th_cond_TLU=[413, 401, 392, 383, 371, 357, 342] W/(K*m)  temp_TLU=[200, 273, 400, 600, 800, 1000, 1200] K  T_specify=off  T_priority=None  T=0 K  T_nominal_specify=off  T_nominal_value=1  T_nominal_unit=K  Q_specify=off  Q_priority=None  Q=0 W  Q_nominal_specify=off  Q_nominal_value=1  Q_nominal_unit=W
  Window : fl_lib/Thermal/Thermal Elements/Thermal Mass  mass_type=foundation.enum.constant_variable.constant  mass=winMaterialMass kg  sp_heat=winMaterialCp J/(K*kg)  mass_min=1e-6 kg  num_ports=foundation.enum.numPorts2.one  m_specify=off  m_priority=High  m=1 kg  m_nominal_specify=off  m_nominal_value=1  m_nominal_unit=kg  T_specify=on  T_priority=High  T=winTemperature K  T_nominal_specify=off  T_nominal_value=1  T_nominal_unit=K  Q_specify=off  Q_priority=None  Q=0 W  Q_nominal_specify=off  Q_nominal_value=1  Q_nominal_unit=W
  WindowAbsorptivity : fl_lib/Physical Signals/Functions/PS Gain  gain=winAbsorptivity
  WindowArea : fl_lib/Physical Signals/Functions/PS Gain  gain=winArea m^2
  WindowHeatToRoom : fl_lib/Thermal/Thermal Elements/Convective Heat Transfer  thermal_type=foundation.enum.constant_variable.constant  area=winArea m^2  heat_tr_coeff=intToRoomHTC W/(K*m^2)  min_heat_tr_coeff=1e-3 W/(K*m^2)  T_specify=off  T_priority=None  T=0 K  T_nominal_specify=off  T_nominal_value=1  T_nominal_unit=K  Q_specify=off  Q_priority=None  Q=0 W  Q_nominal_specify=off  Q_nominal_value=1  Q_nominal_unit=W
  WindowHeatTransferExt : fl_lib/Thermal/Thermal Elements/Conductive Heat Transfer  thermal_type=foundation.enum.ConstantVariableTabulated.Constant  wall_geometry=foundation.enum.ConductionWallGeometry.Planar  area=winArea m^2  thickness=winThickness m  d_in=0.05 m  d_out=0.1 m  L=1 m  th_cond_min=10 W/(K*m)  th_cond=winThermalK W/(K*m)  th_cond_TLU=[413, 401, 392, 383, 371, 357, 342] W/(K*m)  temp_TLU=[200, 273, 400, 600, 800, 1000, 1200] K  T_specify=off  T_priority=None  T=0 K  T_nominal_specify=off  T_nominal_value=1  T_nominal_unit=K  Q_specify=off  Q_priority=None  Q=0 W  Q_nominal_specify=off  Q_nominal_value=1  Q_nominal_unit=W
  WindowHeatTransferInt : fl_lib/Thermal/Thermal Elements/Conductive Heat Transfer  thermal_type=foundation.enum.ConstantVariableTabulated.Constant  wall_geometry=foundation.enum.ConductionWallGeometry.Planar  area=winArea m^2  thickness=winThickness m  d_in=0.05 m  d_out=0.1 m  L=1 m  th_cond_min=10 W/(K*m)  th_cond=winThermalK W/(K*m)  th_cond_TLU=[413, 401, 392, 383, 371, 357, 342] W/(K*m)  temp_TLU=[200, 273, 400, 600, 800, 1000, 1200] K  T_specify=off  T_priority=None  T=0 K  T_nominal_specify=off  T_nominal_value=1  T_nominal_unit=K  Q_specify=off  Q_priority=None  Q=0 W  Q_nominal_specify=off  Q_nominal_value=1  Q_nominal_unit=W
  WindowTransmissivity : fl_lib/Physical Signals/Functions/PS Gain  gain=winTransmissivity
  EXT : PMIOPort  Side=Left
  INT : PMIOPort  Port=2  Side=Right
  SUN : PMIOPort  Port=3  Side=Left
  connections:
  WallHeatToRoom/LConn1 -- WallHeatTransferInt/RConn1
  WindowHeatToRoom/LConn1 -- WindowHeatTransferInt/RConn1
  WindowHeatTransferInt/LConn1 -- WindowHeatTransferExt/RConn1 -- Window/LConn1
  VentAirFlowToRoom/RConn1 -- INT/RConn1 -- SunlightToRoom/LConn1 -- WindowHeatToRoom/RConn1 -- WallHeatToRoom/RConn1
  VentAirFlowToRoom/LConn1 -- SunlightWall/RConn2 -- EXT/RConn1 -- SunlightWindow/RConn2 -- EnvHeatToWindow/LConn1 -- SunlightToRoom/RConn2 -- EnvHeatToWall/LConn1
  WallHeatTransferExt/LConn1 -- SunlightWall/LConn1 -- EnvHeatToWall/RConn1
  WindowHeatTransferExt/LConn1 -- SunlightWindow/LConn1 -- EnvHeatToWindow/RConn1
  WallHeatTransferExt/RConn1 -- WallHeatTransferInt/LConn1 -- SolidWall/LConn1
  WindowAbsorptivity/LConn1 -- WindowTransmissivity/LConn1 -- WindowArea/RConn1
  SunlightToRoom/RConn1 -- WindowTransmissivity/RConn1
  WallAbsorptivity/RConn1 -- SunlightWall/RConn1
  WindowAbsorptivity/RConn1 -- SunlightWindow/RConn1
  WindowArea/LConn1 -- WallArea/LConn1 -- SUN/RConn1
  WallArea/RConn1 -- WallAbsorptivity/LConn1

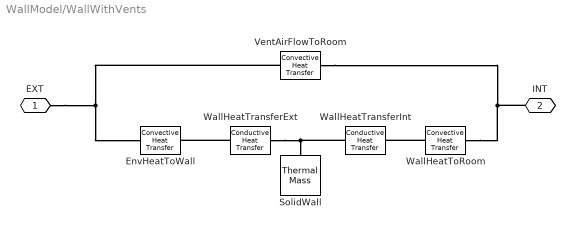
== system WallModel/WallWithVents ==
  EnvHeatToWall : fl_lib/Thermal/Thermal Elements/Convective Heat Transfer  thermal_type=foundation.enum.constant_variable.constant  area=wallArea m^2  heat_tr_coeff=extToWallHTC W/(K*m^2)  min_heat_tr_coeff=1e-3 W/(K*m^2)  T_specify=off  T_priority=None  T=0 K  T_nominal_specify=off  T_nominal_value=1  T_nominal_unit=K  Q_specify=off  Q_priority=None  Q=0 W  Q_nominal_specify=off  Q_nominal_value=1  Q_nominal_unit=W
  SolidWall : fl_lib/Thermal/Thermal Elements/Thermal Mass  mass_type=foundation.enum.constant_variable.constant  mass=wallMaterialMass kg  sp_heat=wallMaterialCp J/(K*kg)  mass_min=1e-6 kg  num_ports=foundation.enum.numPorts2.one  m_specify=off  m_priority=High  m=1 kg  m_nominal_specify=off  m_nominal_value=1  m_nominal_unit=kg  T_specify=on  T_priority=High  T=wallTemperature K  T_nominal_specify=off  T_nominal_value=1  T_nominal_unit=K  Q_specify=off  Q_priority=None  Q=0 W  Q_nominal_specify=off  Q_nominal_value=1  Q_nominal_unit=W
  VentAirFlowToRoom : fl_lib/Thermal/Thermal Elements/Convective Heat Transfer  thermal_type=foundation.enum.constant_variable.constant  area=ventArea m^2  heat_tr_coeff=extToWallHTC W/(K*m^2)  min_heat_tr_coeff=1e-3 W/(K*m^2)  T_specify=off  T_priority=None  T=0 K  T_nominal_specify=off  T_nominal_value=1  T_nominal_unit=K  Q_specify=off  Q_priority=None  Q=0 W  Q_nominal_specify=off  Q_nominal_value=1  Q_nominal_unit=W
  WallHeatToRoom : fl_lib/Thermal/Thermal Elements/Convective Heat Transfer  thermal_type=foundation.enum.constant_variable.constant  area=wallArea m^2  heat_tr_coeff=intToRoomHTC W/(K*m^2)  min_heat_tr_coeff=1e-3 W/(K*m^2)  T_specify=off  T_priority=None  T=0 K  T_nominal_specify=off  T_nominal_value=1  T_nominal_unit=K  Q_specify=off  Q_priority=None  Q=0 W  Q_nominal_specify=off  Q_nominal_value=1  Q_nominal_unit=W
  WallHeatTransferExt : fl_lib/Thermal/Thermal Elements/Conductive Heat Transfer  thermal_type=foundation.enum.ConstantVariableTabulated.Constant  wall_geometry=foundation.enum.ConductionWallGeometry.Planar  area=wallArea m^2  thickness=wallThickness m  d_in=0.05 m  d_out=0.1 m  L=1 m  th_cond_min=10 W/(K*m)  th_cond=wallThermalK W/(K*m)  th_cond_TLU=[413, 401, 392, 383, 371, 357, 342] W/(K*m)  temp_TLU=[200, 273, 400, 600, 800, 1000, 1200] K  T_specify=off  T_priority=None  T=0 K  T_nominal_specify=off  T_nominal_value=1  T_nominal_unit=K  Q_specify=off  Q_priority=None  Q=0 W  Q_nominal_specify=off  Q_nominal_value=1  Q_nominal_unit=W
  WallHeatTransferInt : fl_lib/Thermal/Thermal Elements/Conductive Heat Transfer  thermal_type=foundation.enum.ConstantVariableTabulated.Constant  wall_geometry=foundation.enum.ConductionWallGeometry.Planar  area=wallArea m^2  thickness=wallThickness m  d_in=0.05 m  d_out=0.1 m  L=1 m  th_cond_min=10 W/(K*m)  th_cond=wallThermalK W/(K*m)  th_cond_TLU=[413, 401, 392, 383, 371, 357, 342] W/(K*m)  temp_TLU=[200, 273, 400, 600, 800, 1000, 1200] K  T_specify=off  T_priority=None  T=0 K  T_nominal_specify=off  T_nominal_value=1  T_nominal_unit=K  Q_specify=off  Q_priority=None  Q=0 W  Q_nominal_specify=off  Q_nominal_value=1  Q_nominal_unit=W
  EXT : PMIOPort  Side=Left
  INT : PMIOPort  Port=2  Side=Right
  connections:
  WallHeatToRoom/LConn1 -- WallHeatTransferInt/RConn1
  VentAirFlowToRoom/RConn1 -- WallHeatToRoom/RConn1 -- INT/RConn1
  VentAirFlowToRoom/LConn1 -- EXT/RConn1 -- EnvHeatToWall/LConn1
  WallHeatTransferExt/LConn1 -- EnvHeatToWall/RConn1
  WallHeatTransferExt/RConn1 -- WallHeatTransferInt/LConn1 -- SolidWall/LConn1
